simulink model "sm_tracked_vehicle_belt"  (R2025a)
settings: Solver=ode23t  StartTime=0.0  StopTime=50  MaxStep=0.01  RelTol=1e-4  AbsTol=1e-5  EnableMultiTasking=on
PreLoadFcn:
  | sm_tracked_vehicle_belt_param
StartFcn:
  | tic;
StopFcn:
  | Elapsed_Sim_Time = toc;
  | disp(['Elapsed Sim Time = ' num2str(Elapsed_Sim_Time)]);
undefined symbols (not defined in the file): belt, roller, vehbody, X, Y, Z
libraries: sm_lib x9, nesl_utility x3, SCF_Custom_Forces_lib x2, simulink x2, sm_tracked_vehicle_belt_lib x2, Camera_Frame_Definitions x1
CloseFcn:
  | try,close(h1_sm_tread_drive),end
  | clear h1_sm_tread_drive
  | 
  | clear logsout_sm_tread_drive
  | clear simlog_sm_tread_drive
Description:
  | Tread Drive on Uneven Surface
  | 
  | Copyright 2018-2026 The MathWorks, Inc.
settings Model: Creator=smiller  LastModifiedBy=smiller
settings SolverCC: AutoScaleAbsTol=off  AlgebraicLoopSolver=TrustRegion
settings DataIOCC: SaveFormat=Array  ReturnWorkspaceOutputs=off  SignalLoggingName=logsout_sm_tracked_vehicle_belt
settings OptimizationCC: ReuseModelBlockBuffer=off  LifeSpan=inf
settings DebuggingCC: SolverPrmCheckMsg=warning  UnconnectedInputMsg=warning  UnconnectedLineMsg=warning  AllowSymbolicDim=off  PregeneratedLibrarySubsystemCodeDiagnostic=none  SFUnexpectedBacktrackingDiag=warning  SFNoUnconditionalDefaultTransitionDiag=warning  SFExecutionAtInitializationDiag=none  ArithmeticOperatorsInVariantConditions=warning
settings HardwareCC: ProdBitPerPointer=32.0  ProdBitPerSizeT=32.0  ProdBitPerPtrDiffT=32.0  ProdLargestAtomicFloat=None  ProdIntDivRoundTo=Undefined  ProdEndianess=Unspecified  ProdWordSize=32.0  ProdHWDeviceType=32-bit Generic
settings ModelReferenceCC: EnableRefExpFcnMdlSchedulingChecks=on  PropagateSignalLabelsOutOfModel=off
settings SFSimCC: SimUseLocalCustomCode=off  CustomCodeUndefinedFunction=UseInterfaceOnly
settings RTWCC: RTWUseLocalCustomCode=off  GPUComputeCapability=3.5  DLArmComputeVersion=19.05
settings CodeAppCC: StateflowObjectComments=on
settings GRTTargetCC: TargetLangStandard=C89/C90 (ANSI)
settings ConfigComp: CovMetricSettings=dw  CovSaveCumulativeToWorkspaceVar=on  CovSaveSingleToWorkspaceVar=on  CovExternalEMLEnable=off  CovSFcnEnable=off
settings SimscapeCC: SimscapeNormalizeSystem=off  SimscapeLogType=all  SimscapeLogSimulationStatistics=on  SimscapeLogName=simlog_sm_tracked_vehicle_belt  SimscapeLogLimitData=off  SimscapeLogDataHistory=20000.0
settings ConfigurationSet: Description=SimMechanics 2G
settings DiagnosticsConfigSet: SimMechanicsConflictingReferenceFrames=none  SimMechanicsRigidlyBoundBlock=none
settings ExplorerConfigSet: InternalSimMechanicsExplorerSettings="<ExplorerConfiguration><canonicalview>default</canonicalview><AnimationSetting><BasePlaybackSpeed>1.0</BasePlaybackSpeed><PlaybackSpeedFactor>2.0</PlaybackSpeedFactor></AnimationSetting><TilePanel><TileInfo><Tiles Columns=\"2\" Count=\"3\" Rows=\"2\"><Column Weight=\"0.4996\"/><Column Weight=\"0.5004\"/><Row Weight=\"0.6676\"/><Row Weight=\"0.3324\"/><Tile Height=\"2\" Width=\"1\" X=\"0\" Y=\"0\"/><Tile Height=\"1\" Width=\"1\" X=\"1\" Y=\"0\"/><Tile Height=\"1\" Width=\"1\" X=\"1\" Y=\"1\"/></Tiles></TileInfo><SceneInfo><SceneViewer><BGColor><R>1</R><G>1</G><B>1</B></BGColor><Camera><DoPerspective>on</DoPerspective><Position><X>1.93552410841574951</X><Y>-22.2249086507629947</Y><Z>1.90260789180906764</Z></Position><Center><X>1.18525502751870504</X><Y>-21.5996844166821234</Y><Z>1.68768706134376867</Z></Center><Up><X>-0.16510675539218278</X><Y>0.137588962826818928</Y><Z>0.976631474319820447</Z></Up><ViewLimDist>1</ViewLimDist><YLim>0.466307658154998583</YLim><XLim>0.425934700738981431</XLim></Camera></SceneViewer><SceneViewer><BGColor><R>1</R><G>1</G><B>1</B></BGColor><Camera><DoPerspective>off</DoPerspective><Position><X>9.13279417173888497</X><Y>-10.8073529611331143</Y><Z>295.016351338458605</Z></Position><Center><X>9.13279417173888497</X><Y>-10.8073529611331143</Y><Z>-0.0192398869523913163</Z></Center><Up><X>0</X><Y>1</Y><Z>-0</Z></Up><ViewLimDist>1</ViewLimDist><YLim>13.4087479739997679</YLim><XLim>18.561454619030247</XLim></Camera></SceneViewer><SceneViewer><BGColor><R>1</R><G>1</G><B>1</B></BGColor><Camera><DoPerspective>on</DoPerspective><Position><X>3.00605602641301672</X><Y>-17.9535217836110448</Y><Z>1.77667486241447481</Z></Position><Center><X>2.04688726115486386</X><Y>-18.1627945947119365</Y><Z>1.58641143900608261</Z></Center><Up><X>-0.185488496866644897</X><Y>-0.0423982058506443826</Y><Z>0.981731332733553508</Z></Up><ViewLimDist>1</ViewLimDist><YLim>0.466307658154998583</YLim><XLim>1.30813741270030581</XLim></Camera></SceneViewer></SceneInfo></TilePanel><MechEditorPanel><Cameras><Camera><Id>Camera1</Id><Value><Name>Track FixO FR</Name><NativeCamera><PositionTrackingFeature>Camera_Frames.Frame_FixO_FR.R</PositionTrackingFeature><CenterTrackingFeature>Camera_Frames.Frame_FixO_FR.R</CenterTrackingFeature><UpVectorTrackingFeature>Camera_Frames.Frame_FixO_FR.R</UpVectorTrackingFeature><CenterTrackingOrigin>off</CenterTrackingOrigin><CenterTrackingDirection>+X</CenterTrackingDirection><UpVectorTrackingDirection>+Z</UpVectorTrackingDirection></NativeCamera></Value></Camera><Camera><Id>Camera2</Id><Value><Name>Track FixO Right</Name><NativeCamera><PositionTrackingFeature>Camera_Frames.Frame_FixO_Right.R</PositionTrackingFeature><CenterTrackingFeature>Camera_Frames.Frame_FixO_Right.R</CenterTrackingFeature><UpVectorTrackingFeature>Camera_Frames.Frame_FixO_Right.R</UpVectorTrackingFeature><CenterTrackingOrigin>off</CenterTrackingOrigin><CenterTrackingDirection>+X</CenterTrackingDirection><UpVectorTrackingDirection>+Z</UpVectorTrackingDirection></NativeCamera></Value></Camera><Camera><Id>Camera3</Id><Value><Name>Track FixO RR</Name><NativeCamera><PositionTrackingFeature>Camera_Frames.Frame_FixO_RR.R</PositionTrackingFeature><CenterTrackingFeature>Camera_Frames.Frame_FixO_RR.R</CenterTrackingFeature><UpVectorTrackingFeature>Camera_Frames.Frame_FixO_RR.R</UpVectorTrackingFeature><CenterTrackingOrigin>off</CenterTrackingOrigin><CenterTrackingDirection>+X</CenterTrackingDirection><UpVectorTrackingDirection>+Z</UpVectorTrackingDirection></NativeCamera></Value></Camera><Camera><Id>Camera4</Id><Value><Name>Track FixO RL</Name><NativeCamera><PositionTrackingFeature>Camera_Frames.Frame_FixO_RL.R</PositionTrackingFeature><CenterTrackingFeature>Camera_Frames.Frame_FixO_RL.R</CenterTrackingFeature><UpVectorTrackingFeature>Camera_Frames.Frame_FixO_RL.R</UpVectorTrackingFeature><CenterTrackingOrigin>off</CenterTrackingOrigin><CenterTrackingDirection>+X</CenterTrackingDirection><UpVectorTrackingDirection>+Z</UpVectorTrackingDirection></NativeCamera></Value></Camera><Camera><Id>Camera5</Id><Value><Name>Track FixO Left</Name><NativeCamera><PositionTrackingFeature>Camera_Frames.Frame_FixO_Left.R</PositionTrackingFeature><CenterTrackingFeature>Camera_Frames.Frame_FixO_Left.R</CenterTrackingFeature><UpVectorTrackingFeature>Camera_Frames.Frame_FixO_Left.R</UpVectorTrackingFeature><CenterTrackingOrigin>off</CenterTrackingOrigin><CenterTrackingDirection>+X</CenterTrackingDirection><UpVectorTrackingDirection>+Z</UpVectorTrackingDirection></NativeCamera></Value></Camera><Camera><Id>Camera6</Id><Value><Name>Track FixO FL</Name><NativeCamera><PositionTrackingFeature>Camera_Frames.Frame_FixO_FL.R</PositionTrackingFeature><CenterTrackingFeature>Camera_Frames.Frame_FixO_FL.R</CenterTrackingFeature><UpVectorTrackingFeature>Camera_Frames.Frame_FixO_FL.R</UpVectorTrackingFeature><CenterTrackingOrigin>off</CenterTrackingOrigin><CenterTrackingDirection>+X</CenterTrackingDirection><UpVectorTrackingDirection>+Z</UpVectorTrackingDirection></NativeCamera></Value></Camera><Camera><Id>Camera7</Id><Value><Name>Track FixO Top</Name><NativeCamera><PositionTrackingFeature>Camera_Frames.Frame_FixO_Top.R</PositionTrackingFeature><CenterTrackingFeature>Camera_Frames.Frame_FixO_Top.R</CenterTrackingFeature><UpVectorTrackingFeature>Camera_Frames.Frame_FixO_Top.R</UpVectorTrackingFeature><CenterTrackingOrigin>off</CenterTrackingOrigin><CenterTrackingDirection>+X</CenterTrackingDirection><UpVectorTrackingDirection>+Z</UpVectorTrackingDirection></NativeCamera></Value></Camera><Camera><Id>Camera8</Id><Value><Name>Track FixO Front</Name><NativeCamera><PositionTrackingFeature>Camera_Frames.Frame_FixO_Front.R</PositionTrackingFeature><CenterTrackingFeature>Camera_Frames.Frame_FixO_Front.R</CenterTrackingFeature><UpVectorTrackingFeature>Camera_Frames.Frame_FixO_Front.R</UpVectorTrackingFeature><CenterTrackingOrigin>off</CenterTrackingOrigin><CenterTrackingDirection>+X</CenterTrackingDirection><UpVectorTrackingDirection>+Z</UpVectorTrackingDirection></NativeCamera></Value></Camera><Camera><Id>Camera9</Id><Value><Name>Track FixO Rear</Name><NativeCamera><PositionTrackingFeature>Camera_Frames.Frame_FixO_Rear.R</PositionTrackingFeature><CenterTrackingFeature>Camera_Frames.Frame_FixO_Rear.R</CenterTrackingFeature><UpVectorTrackingFeature>Camera_Frames.Frame_FixO_Rear.R</UpVectorTrackingFeature><CenterTrackingOrigin>off</CenterTrackingOrigin><CenterTrackingDirection>+X</CenterTrackingDirection><UpVectorTrackingDirection>+Z</UpVectorTrackingDirection></NativeCamera></Value></Camera><Camera><Id>Camera10</Id><Value><Name>Track FR</Name><NativeCamera><PositionTrackingFeature>Camera_Frames.Frame_FR.R</PositionTrackingFeature><CenterTrackingFeature>Camera_Frames.Frame_FR.R</CenterTrackingFeature><UpVectorTrackingFeature>Camera_Frames.Frame_FR.R</UpVectorTrackingFeature><CenterTrackingOrigin>off</CenterTrackingOrigin><CenterTrackingDirection>+X</CenterTrackingDirection><UpVectorTrackingDirection>+Z</UpVectorTrackingDirection></NativeCamera></Value></Camera><Camera><Id>Camera11</Id><Value><Name>Track Right</Name><NativeCamera><PositionTrackingFeature>Camera_Frames.Frame_Right.R</PositionTrackingFeature><CenterTrackingFeature>Camera_Frames.Frame_Right.R</CenterTrackingFeature><UpVectorTrackingFeature>Camera_Frames.Frame_Right.R</UpVectorTrackingFeature><CenterTrackingOrigin>off</CenterTrackingOrigin><CenterTrackingDirection>+X</CenterTrackingDirection><UpVectorTrackingDirection>+Z</UpVectorTrackingDirection></NativeCamera></Value></Camera><Camera><Id>Camera12</Id><Value><Name>Track RR</Name><NativeCamera><PositionTrackingFeature>Camera_Frames.Frame_RR.R</PositionTrackingFeature><CenterTrackingFeature>Camera_Frames.Frame_RR.R</CenterTrackingFeature><UpVectorTrackingFeature>Camera_Frames.Frame_RR.R</UpVectorTrackingFeature><CenterTrackingOrigin>off</CenterTrackingOrigin><CenterTrackingDirection>+X</CenterTrackingDirection><UpVectorTrackingDirection>+Z</UpVectorTrackingDirection></NativeCamera></Value></Camera><Camera><Id>Camera13</Id><Value><Name>Track RL</Name><NativeCamera><PositionTrackingFeature>Camera_Frames.Frame_RL.R</PositionTrackingFeature><CenterTrackingFeature>Camera_Frames.Frame_RL.R</CenterTrackingFeature><UpVectorTrackingFeature>Camera_Frames.Frame_RL.R</UpVectorTrackingFeature><CenterTrackingOrigin>off</CenterTrackingOrigin><CenterTrackingDirection>+X</CenterTrackingDirection><UpVectorTrackingDirection>+Z</UpVectorTrackingDirection></NativeCamera></Value></Camera><Camera><Id>Camera14</Id><Value><Name>Track Left</Name><NativeCamera><PositionTrackingFeature>Camera_Frames.Frame_Left.R</PositionTrackingFeature><CenterTrackingFeature>Camera_Frames.Frame_Left.R</CenterTrackingFeature><UpVectorTrackingFeature>Camera_Frames.Frame_Left.R</UpVectorTrackingFeature><CenterTrackingOrigin>off</CenterTrackingOrigin><CenterTrackingDirection>+X</CenterTrackingDirection><UpVectorTrackingDirection>+Z</UpVectorTrackingDirection></NativeCamera></Value></Camera><Camera><Id>Camera15</Id><Value><Name>Track FL</Name><NativeCamera><PositionTrackingFeature>Camera_Frames.Frame_FL.R</PositionTrackingFeature><CenterTrackingFeature>Camera_Frames.Frame_FL.R</CenterTrackingFeature><UpVectorTrackingFeature>Camera_Frames.Frame_FL.R</UpVectorTrackingFeature><CenterTrackingOrigin>off</CenterTrackingOrigin><CenterTrackingDirection>+X</CenterTrackingDirection><UpVectorTrackingDirection>+Z</UpVectorTrackingDirection></NativeCamera></Value></Camera><Camera><Id>Camera16</Id><Value><Name>Track Top</Name><NativeCamera><PositionTrackingFeature>Camera_Frames.Frame_Top.R</PositionTrackingFeature><CenterTrackingFeature>Camera_Frames.Frame_Top.R</CenterTrackingFeature><UpVectorTrackingFeature>Camera_Frames.Frame_Top.R</UpVectorTrackingFeature><CenterTrackingOrigin>off</CenterTrackingOrigin><CenterTrackingDirection>+X</CenterTrackingDirection><UpVectorTrackingDirection>+Z</UpVectorTrackingDirection></NativeCamera></Value></Camera><Camera><Id>Camera17</Id><Value><Name>Track Front</Name><NativeCamera><PositionTrackingFeature>Camera_Frames.Frame_Front.R</PositionTrackingFeature><CenterTrackingFeature>Camera_Frames.Frame_Front.R</CenterTrackingFeature><UpVectorTrackingFeature>Camera_Frames.Frame_Front.R</UpVectorTrackingFeature><CenterTrackingOrigin>off</CenterTrackingOrigin><CenterTrackingDirection>+X</CenterTrackingDirection><UpVectorTrackingDirection>+Z</UpVectorTrackingDirection></NativeCamera></Value></Camera><Camera><Id>Camera18</Id><Value><Name>Track Rear</Name><NativeCamera><PositionTrackingFeature>Camera_Frames.Frame_Rear.R</PositionTrackingFeature><CenterTrackingFeature>Camera_Frames.Frame_Rear.R</CenterTrackingFeature><UpVectorTrackingFeature>Camera_Frames.Frame_Rear.R</UpVectorTrackingFeature><CenterTrackingOrigin>off</CenterTrackingOrigin><CenterTrackingDirection>+X</CenterTrackingDirection><UpVectorTrackingDirection>+Z</UpVectorTrackingDirection></NativeCamera></Value></Camera><Camera><Id>Camera19</Id><Value><Name>Track SuspF</Name><NativeCamera><PositionTrackingFeature>Camera_Frames.Frame_SuspF.R</PositionTrackingFeature><CenterTrackingFeature>Camera_Frames.Frame_SuspF.R</CenterTrackingFeature><UpVectorTrackingFeature>Camera_Frames.Frame_SuspF.R</UpVectorTrackingFeature><CenterTrackingOrigin>off</CenterTrackingOrigin><CenterTrackingDirection>+X</CenterTrackingDirection><UpVectorTrackingDirection>+Z</UpVectorTrackingDirection></NativeCamera></Value></Camera><Camera><Id>Camera20</Id><Value><Name>Track SuspR</Name><NativeCamera><PositionTrackingFeature>Camera_Frames.Frame_SuspR.R</PositionTrackingFeature><CenterTrackingFeature>Camera_Frames.Frame_SuspR.R</CenterTrackingFeature><UpVectorTrackingFeature>Camera_Frames.Frame_SuspR.R</UpVectorTrackingFeature><CenterTrackingOrigin>off</CenterTrackingOrigin><CenterTrackingDirection>+X</CenterTrackingDirection><UpVectorTrackingDirection>+Z</UpVectorTrackingDirection></NativeCamera></Value></Camera><Camera><Id>Camera21</Id><Value><Name>Track WheelFR</Name><NativeCamera><PositionTrackingFeature>Camera_Frames.Frame_Wheel_FR.R</PositionTrackingFeature><CenterTrackingFeature>Camera_Frames.Frame_Wheel_FR.R</CenterTrackingFeature><UpVectorTrackingFeature>Camera_Frames.Frame_Wheel_FR.R</UpVectorTrackingFeature><CenterTrackingOrigin>off</CenterTrackingOrigin><CenterTrackingDirection>+X</CenterTrackingDirection><UpVectorTrackingDirection>+Z</UpVectorTrackingDirection></NativeCamera></Value></Camera><Camera><Id>Camera22</Id><Value><Name>Track WheelRR</Name><NativeCamera><PositionTrackingFeature>Camera_Frames.Frame_Wheel_RR.R</PositionTrackingFeature><CenterTrackingFeature>Camera_Frames.Frame_Wheel_RR.R</CenterTrackingFeature><UpVectorTrackingFeature>Camera_Frames.Frame_Wheel_RR.R</UpVectorTrackingFeature><CenterTrackingOrigin>off</CenterTrackingOrigin><CenterTrackingDirection>+X</CenterTrackingDirection><UpVectorTrackingDirection>+Z</UpVectorTrackingDirection></NativeCamera></Value></Camera><Camera><Id>Camera23</Id><Value><Name>Track WheelRL</Name><NativeCamera><PositionTrackingFeature>Camera_Frames.Frame_Wheel_RL.R</PositionTrackingFeature><CenterTrackingFeature>Camera_Frames.Frame_Wheel_RL.R</CenterTrackingFeature><UpVectorTrackingFeature>Camera_Frames.Frame_Wheel_RL.R</UpVectorTrackingFeature><CenterTrackingOrigin>off</CenterTrackingOrigin><CenterTrackingDirection>+X</CenterTrackingDirection><UpVectorTrackingDirection>+Z</UpVectorTrackingDirection></NativeCamera></Value></Camera><Camera><Id>Camera24</Id><Value><Name>Track WheelFL</Name><NativeCamera><PositionTrackingFeature>Camera_Frames.Frame_Wheel_FL.R</PositionTrackingFeature><CenterTrackingFeature>Camera_Frames.Frame_Wheel_FL.R</CenterTrackingFeature><UpVectorTrackingFeature>Camera_Frames.Frame_Wheel_FL.R</UpVectorTrackingFeature><CenterTrackingOrigin>off</CenterTrackingOrigin><CenterTrackingDirection>+X</CenterTrackingDirection><UpVectorTrackingDirection>+Z</UpVectorTrackingDirection></NativeCamera></Value></Camera><Camera><Id>Camera25</Id><Value><Name>View Seat FL</Name><NativeCamera><PositionTrackingFeature>Camera_Frames.Frame_View_Seat_FL.R</PositionTrackingFeature><CenterTrackingFeature>Camera_Frames.Frame_View_Seat_FL.R</CenterTrackingFeature><UpVectorTrackingFeature>Camera_Frames.Frame_View_Seat_FL.R</UpVectorTrackingFeature><CenterTrackingOrigin>off</CenterTrackingOrigin><CenterTrackingDirection>+X</CenterTrackingDirection><UpVectorTrackingDirection>+Z</UpVectorTrackingDirection></NativeCamera></Value></Camera><Camera><Id>Camera26</Id><Value><Name>View Seat FR</Name><NativeCamera><PositionTrackingFeature>Camera_Frames.Frame_View_Seat_FR.R</PositionTrackingFeature><CenterTrackingFeature>Camera_Frames.Frame_View_Seat_FR.R</CenterTrackingFeature><UpVectorTrackingFeature>Camera_Frames.Frame_View_Seat_FR.R</UpVectorTrackingFeature><CenterTrackingOrigin>off</CenterTrackingOrigin><CenterTrackingDirection>+X</CenterTrackingDirection><UpVectorTrackingDirection>+Z</UpVectorTrackingDirection></NativeCamera></Value></Camera><Camera><Id>Camera27</Id><Value><Name>View Susp FR</Name><NativeCamera><PositionTrackingFeature>Camera_Frames.Frame_View_Susp_FR.R</PositionTrackingFeature><CenterTrackingFeature>Camera_Frames.Frame_View_Susp_FR.R</CenterTrackingFeature><UpVectorTrackingFeature>Camera_Frames.Frame_View_Susp_FR.R</UpVectorTrackingFeature><CenterTrackingOrigin>off</CenterTrackingOrigin><CenterTrackingDirection>+X</CenterTrackingDirection><UpVectorTrackingDirection>+Z</UpVectorTrackingDirection></NativeCamera></Value></Camera><Camera><Id>Camera28</Id><Value><Name>View Susp RR</Name><NativeCamera><PositionTrackingFeature>Camera_Frames.Frame_View_Susp_RR.R</PositionTrackingFeature><CenterTrackingFeature>Camera_Frames.Frame_View_Susp_RR.R</CenterTrackingFeature><UpVectorTrackingFeature>Camera_Frames.Frame_View_Susp_RR.R</UpVectorTrackingFeature><CenterTrackingOrigin>off</CenterTrackingOrigin><CenterTrackingDirection>+X</CenterTrackingDirection><UpVectorTrackingDirection>+Z</UpVectorTrackingDirection></NativeCamera></Value></Camera><Camera><Id>Camera29</Id><Value><Name>View Susp RL</Name><NativeCamera><PositionTrackingFeature>Camera_Frames.Frame_View_Susp_RL.R</PositionTrackingFeature><CenterTrackingFeature>Camera_Frames.Frame_View_Susp_RL.R</CenterTrackingFeature><UpVectorTrackingFeature>Camera_Frames.Frame_View_Susp_RL.R</UpVectorTrackingFeature><CenterTrackingOrigin>off</CenterTrackingOrigin><CenterTrackingDirection>+X</CenterTrackingDirection><UpVectorTrackingDirection>+Z</UpVectorTrackingDirection></NativeCamera></Value></Camera><Camera><Id>Camera30</Id><Value><Name>View Susp FL</Name><NativeCamera><PositionTrackingFeature>Camera_Frames.Frame_View_Susp_FL.R</PositionTrackingFeature><CenterTrackingFeature>Camera_Frames.Frame_View_Susp_FL.R</CenterTrackingFeature><UpVectorTrackingFeature>Camera_Frames.Frame_View_Susp_FL.R</UpVectorTrackingFeature><CenterTrackingOrigin>off</CenterTrackingOrigin><CenterTrackingDirection>+X</CenterTrackingDirection><UpVectorTrackingDirection>+Z</UpVectorTrackingDirection></NativeCamera></Value></Camera><Camera><Id>Camera31</Id><Value><Name>Dolly Camera</Name><NativeCamera><PositionTrackingFeature>Camera_Frames.Frame_Dolly.R</PositionTrackingFeature><CenterTrackingFeature>Camera_Frames.Frame_Dolly.R</CenterTrackingFeature><UpVectorTrackingFeature>Camera_Frames.Frame_Dolly.R</UpVectorTrackingFeature><CenterTrackingOrigin>off</CenterTrackingOrigin><CenterTrackingDirection>+X</CenterTrackingDirection><UpVectorTrackingDirection>+Z</UpVectorTrackingDirection></NativeCamera></Value></Camera><Camera><Id>Camera32</Id><Value><Name>Track Dolly Camera</Name><NativeCamera><PositionTrackingFeature>Camera_Frames.Frame_Dolly.R</PositionTrackingFeature><CenterTrackingFeature>Camera_Frames.Transform_Camera_Ref.F</CenterTrackingFeature><UpVectorTrackingFeature>Camera_Frames.World_Frame.W</UpVectorTrackingFeature><CenterTrackingOrigin>on</CenterTrackingOrigin><UpVectorTrackingDirection>+Z</UpVectorTrackingDirection></NativeCamera></Value></Camera></Cameras><GfxPanelCameraMap><MapElement CameraMLId=\"Camera1\" GfxPanelIndex=\"0\"/><MapElement CameraMLId=\"Camera18\" GfxPanelIndex=\"2\"/></GfxPanelCameraMap><VideoCreator><PlaybackSpeedRatio>1.0</PlaybackSpeedRatio><FrameRate>30</FrameRate><VideoFormat>MPEG-4</VideoFormat><FrameSize>[800 450]</FrameSize></VideoCreator></MechEditorPanel></ExplorerConfiguration>"

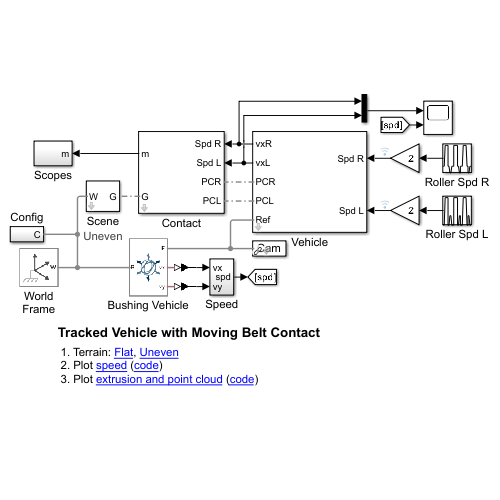
[thumbnail: Simulink's stored preview of the top-level diagram]
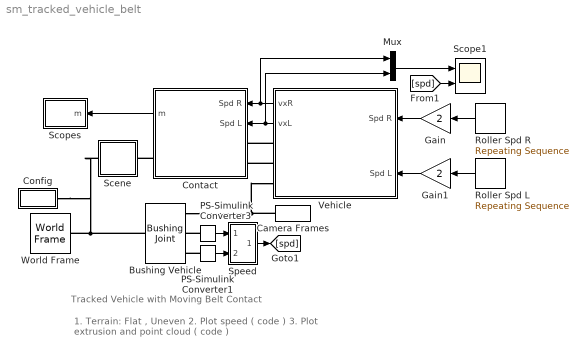
== system sm_tracked_vehicle_belt ==
  note: 1. Terrain: Flat , Uneven
      | 2. Plot speed ( code )
      | 3. Plot extrusion and point cloud ( code )
  note: Tracked Vehicle with Moving Belt Contact
  Bushing Vehicle : sm_lib/Joints/Bushing Joint  JointMode=Normal  CompositeWrenchDir=FollowerOnBase  CompositeWrenchFrame=BaseFrame  SenseConstraintForce=off  SenseConstraintTorque=off  SenseTotalForce=off  SenseTotalTorque=off  PxPositionTargetSpecify=on  PxPositionTargetPriority=High  PxPositionTargetValue=vehbody.x0  PxPositionTargetValueUnits=m  PxVelocityTargetSpecify=off  PxVelocityTargetPriority=High  PxVelocityTargetValue=0  PxVelocityTargetValueUnits=m/s  PxEquilibriumPosition=0  PxEquilibriumPositionUnits=m  PxSpringStiffness=0  PxSpringStiffnessUnits=N/m  PxDampingCoefficient=1  PxDampingCoefficientUnits=N/(m/s)  PxLowerLimitSpecify=off  PxLowerLimitBound=-1  PxLowerLimitBoundUnits=m  PxLowerLimitStiffness=1e6  PxLowerLimitStiffnessUnits=N/m  PxLowerLimitDamping=1e3  PxLowerLimitDampingUnits=N/(m/s)  PxLowerLimitTransitionRegionWidth=1e-4  PxLowerLimitTransitionRegionWidthUnits=m  PxUpperLimitSpecify=off  PxUpperLimitBound=1  PxUpperLimitBoundUnits=m  PxUpperLimitStiffness=1e6  PxUpperLimitStiffnessUnits=N/m  PxUpperLimitDamping=1e3  PxUpperLimitDampingUnits=N/(m/s)  PxUpperLimitTransitionRegionWidth=1e-4  PxUpperLimitTransitionRegionWidthUnits=m  PxTorqueActuationMode=NoTorque  PxMotionActuationMode=ComputedMotion  PxSensePosition=off  PxSenseVelocity=on  PxSenseAcceleration=off  PxSenseTorqueForce=off  PxSenseLowerLimitTorqueForce=off  PxSenseUpperLimitTorqueForce=off  PyPositionTargetSpecify=on  PyPositionTargetPriority=High  PyPositionTargetValue=0  PyPositionTargetValueUnits=m  PyVelocityTargetSpecify=off  PyVelocityTargetPriority=High  PyVelocityTargetValue=0  PyVelocityTargetValueUnits=m/s  PyEquilibriumPosition=0  PyEquilibriumPositionUnits=m  PySpringStiffness=0  PySpringStiffnessUnits=N/m  PyDampingCoefficient=1  PyDampingCoefficientUnits=N/(m/s)  PyLowerLimitSpecify=off  PyLowerLimitBound=-1  PyLowerLimitBoundUnits=m  PyLowerLimitStiffness=1e6  PyLowerLimitStiffnessUnits=N/m  PyLowerLimitDamping=1e3  PyLowerLimitDampingUnits=N/(m/s)  PyLowerLimitTransitionRegionWidth=1e-4  PyLowerLimitTransitionRegionWidthUnits=m  PyUpperLimitSpecify=off  PyUpperLimitBound=1  PyUpperLimitBoundUnits=m  PyUpperLimitStiffness=1e6  PyUpperLimitStiffnessUnits=N/m  PyUpperLimitDamping=1e3  PyUpperLimitDampingUnits=N/(m/s)  PyUpperLimitTransitionRegionWidth=1e-4  PyUpperLimitTransitionRegionWidthUnits=m  PyTorqueActuationMode=NoTorque  PyMotionActuationMode=ComputedMotion  PySensePosition=off  PySenseVelocity=on  PySenseAcceleration=off  PySenseTorqueForce=off  PySenseLowerLimitTorqueForce=off  PySenseUpperLimitTorqueForce=off  PzPositionTargetSpecify=on  PzPositionTargetPriority=High  PzPositionTargetValue=vehbody.z0  PzPositionTargetValueUnits=m  PzVelocityTargetSpecify=off  PzVelocityTargetPriority=High  PzVelocityTargetValue=0  PzVelocityTargetValueUnits=m/s  PzEquilibriumPosition=0  PzEquilibriumPositionUnits=m  PzSpringStiffness=0  PzSpringStiffnessUnits=N/m  PzDampingCoefficient=0  PzDampingCoefficientUnits=N/(m/s)  PzLowerLimitSpecify=off  PzLowerLimitBound=-1  PzLowerLimitBoundUnits=m  PzLowerLimitStiffness=1e6  PzLowerLimitStiffnessUnits=N/m  PzLowerLimitDamping=1e3  PzLowerLimitDampingUnits=N/(m/s)  PzLowerLimitTransitionRegionWidth=1e-4  PzLowerLimitTransitionRegionWidthUnits=m  PzUpperLimitSpecify=off  PzUpperLimitBound=1  PzUpperLimitBoundUnits=m  PzUpperLimitStiffness=1e6  PzUpperLimitStiffnessUnits=N/m  PzUpperLimitDamping=1e3  PzUpperLimitDampingUnits=N/(m/s)  PzUpperLimitTransitionRegionWidth=1e-4  PzUpperLimitTransitionRegionWidthUnits=m  PzTorqueActuationMode=NoTorque  PzMotionActuationMode=ComputedMotion  PzSensePosition=off  PzSenseVelocity=off  PzSenseAcceleration=off  PzSenseTorqueForce=off  PzSenseLowerLimitTorqueForce=off  PzSenseUpperLimitTorqueForce=off  RxPositionTargetSpecify=on  RxPositionTargetPriority=High  RxPositionTargetValue=0  RxPositionTargetValueUnits=deg  RxVelocityTargetSpecify=off  RxVelocityTargetPriority=High  RxVelocityTargetValue=0  RxVelocityTargetValueUnits=deg/s  RxEquilibriumPosition=0  RxEquilibriumPositionUnits=deg  RxSpringStiffness=0  RxSpringStiffnessUnits=N*m/deg  RxDampingCoefficient=0  RxDampingCoefficientUnits=N*m/(deg/s)  RxLowerLimitSpecify=off  RxLowerLimitBound=-90  RxLowerLimitBoundUnits=deg  RxLowerLimitStiffness=1e4  RxLowerLimitStiffnessUnits=N*m/deg  RxLowerLimitDamping=10  RxLowerLimitDampingUnits=N*m/(deg/s)  RxLowerLimitTransitionRegionWidth=0.1  RxLowerLimitTransitionRegionWidthUnits=deg  RxUpperLimitSpecify=off  RxUpperLimitBound=90  RxUpperLimitBoundUnits=deg  RxUpperLimitStiffness=1e4  RxUpperLimitStiffnessUnits=N*m/deg  RxUpperLimitDamping=10  RxUpperLimitDampingUnits=N*m/(deg/s)  RxUpperLimitTransitionRegionWidth=0.1  RxUpperLimitTransitionRegionWidthUnits=deg  RxTorqueActuationMode=NoTorque  RxMotionActuationMode=ComputedMotion  RxSensePosition=off  RxSenseVelocity=off  RxSenseAcceleration=off  RxSenseTorqueForce=off  RxSenseLowerLimitTorqueForce=off  RxSenseUpperLimitTorqueForce=off  RyPositionTargetSpecify=on  RyPositionTargetPriority=High  RyPositionTargetValue=0  RyPositionTargetValueUnits=deg  RyVelocityTargetSpecify=off  RyVelocityTargetPriority=High  RyVelocityTargetValue=0  RyVelocityTargetValueUnits=deg/s  RyEquilibriumPosition=0  RyEquilibriumPositionUnits=deg  RySpringStiffness=0  RySpringStiffnessUnits=N*m/deg  RyDampingCoefficient=0  RyDampingCoefficientUnits=N*m/(deg/s)  RyLowerLimitSpecify=off  RyLowerLimitBound=-90  RyLowerLimitBoundUnits=deg  RyLowerLimitStiffness=1e4  RyLowerLimitStiffnessUnits=N*m/deg  RyLowerLimitDamping=10  RyLowerLimitDampingUnits=N*m/(deg/s)  RyLowerLimitTransitionRegionWidth=0.1  RyLowerLimitTransitionRegionWidthUnits=deg  RyUpperLimitSpecify=off  RyUpperLimitBound=90  RyUpperLimitBoundUnits=deg  RyUpperLimitStiffness=1e4  RyUpperLimitStiffnessUnits=N*m/deg  RyUpperLimitDamping=10  RyUpperLimitDampingUnits=N*m/(deg/s)  RyUpperLimitTransitionRegionWidth=0.1  RyUpperLimitTransitionRegionWidthUnits=deg  RyTorqueActuationMode=NoTorque  RyMotionActuationMode=ComputedMotion  RySensePosition=off  RySenseVelocity=off  RySenseAcceleration=off  RySenseTorqueForce=off  RySenseLowerLimitTorqueForce=off  RySenseUpperLimitTorqueForce=off  RzPositionTargetSpecify=off  RzPositionTargetPriority=High  RzPositionTargetValue=0  RzPositionTargetValueUnits=deg  RzVelocityTargetSpecify=off  RzVelocityTargetPriority=High  RzVelocityTargetValue=0  RzVelocityTargetValueUnits=deg/s  RzEquilibriumPosition=0  RzEquilibriumPositionUnits=deg  RzSpringStiffness=0  RzSpringStiffnessUnits=N*m/deg  RzDampingCoefficient=0  RzDampingCoefficientUnits=N*m/(deg/s)  RzLowerLimitSpecify=off  RzLowerLimitBound=-90  RzLowerLimitBoundUnits=deg  RzLowerLimitStiffness=1e4  RzLowerLimitStiffnessUnits=N*m/deg  RzLowerLimitDamping=10  RzLowerLimitDampingUnits=N*m/(deg/s)  RzLowerLimitTransitionRegionWidth=0.1  RzLowerLimitTransitionRegionWidthUnits=deg  RzUpperLimitSpecify=off  RzUpperLimitBound=90  RzUpperLimitBoundUnits=deg  RzUpperLimitStiffness=1e4  RzUpperLimitStiffnessUnits=N*m/deg  RzUpperLimitDamping=10  RzUpperLimitDampingUnits=N*m/(deg/s)  RzUpperLimitTransitionRegionWidth=0.1  RzUpperLimitTransitionRegionWidthUnits=deg  RzTorqueActuationMode=NoTorque  RzMotionActuationMode=ComputedMotion  RzSensePosition=off  RzSenseVelocity=off  RzSenseAcceleration=off  RzSenseTorqueForce=off  RzSenseLowerLimitTorqueForce=off  RzSenseUpperLimitTorqueForce=off
  Camera Frames : Camera_Frame_Definitions/Camera Frames  Camera=Camera  popup_dolly_camera=XYZ
  Config : Subsystem
  Contact : Subsystem  mask(Contact Forces, Belts to Ground){k_collision=belt.ground.k, d_collision=belt.ground.b, d_width=belt.ground.twd, muk=belt.ground.muk, mus=belt.ground.mus, vth=belt.ground.vth}
      mask prompts: k_collision "Stiffness Coefficient (N/m)"; d_collision "Damping Coefficient (N/(m/s))"; d_width "Transition Region Width (m)"; muk "Coefficient of Kinetic Friction"; mus "Coefficient of Static Friction"; vth "Velocity Threshold"
      mask help: Models contact force between belts and ground. Translational speed of belt is an input to a custom force law that enables the belts to pull themselves across the surface.
      mask TypeOptions k_collision: Contact Track L/k_collision | Contact Track R/k_collision
      mask TypeOptions d_collision: Contact Track L/d_collision | Contact Track R/d_collision
      mask TypeOptions d_width: Contact Track L/d_width | Contact Track R/d_width
      mask TypeOptions muk: Contact Track L/muk | Contact Track R/muk
      mask TypeOptions mus: Contact Track L/mus | Contact Track R/mus
      mask TypeOptions vth: Contact Track L/vth | Contact Track R/vth
      mask DialogControl cont_normalForce Prompt: Normal Force
      mask DialogControl cont_frictionForce Prompt: Friction Force
  Gain : Gain  Gain=2
  Gain1 : Gain  Gain=2
  Mux : Mux  Inputs=2
  PS-Simulink Converter1 : nesl_utility/PS-Simulink Converter  PhysicalDomain=network_engine_domain  SubClassName=ps_output  LeftPortType=input  RightPortType=output  PseudoPeriodic=off  Frequencies=[]  VectorFormat=1-D array  Unit=1  AffineConversion=off
  PS-Simulink Converter3 : nesl_utility/PS-Simulink Converter  PhysicalDomain=network_engine_domain  SubClassName=ps_output  LeftPortType=input  RightPortType=output  PseudoPeriodic=off  Frequencies=[]  VectorFormat=1-D array  Unit=1  AffineConversion=off
  Roller Spd L : simulink/Sources/Repeating Sequence  rep_seq_t=[0 1 1.5 4.5 5 6 6.5 7.5 8 9]  rep_seq_y=[0 0 3 3 0 0 1 1 0 0]
  Roller Spd R : simulink/Sources/Repeating Sequence  rep_seq_t=[0 1 1.5 4.5 5 6 6.5 7.5 8 9]  rep_seq_y=[0 0 3 3 0 0 -1 -1 0 0]
  Scene : Subsystem  mask{popup_terrain=Uneven}
      mask prompts: popup_terrain "Terrain"
      mask init:
      | bh = gcb;
      | if(popup_terrain == 1)
      |     set_param([bh '/Grid Surface'],'ZHeights','Scene.Terrain.z_heights_data*0')
      | else
      |     set_param([bh '/Grid Surface'],'ZHeights','Scene.Terrain.z_heights_data')
      | end
      settings: AttributesFormatString=%<popup_terrain>
      mask TypeOptions popup_terrain: Flat | Uneven
  Scope1 : Scope  NumInputPorts=2
      settings: ActiveDisplayYMinimum=-0.88266  ActiveDisplayYMaximum=2.06398
  Scopes : Subsystem
  Speed : Subsystem
  Vehicle : Subsystem  mask{cyl_radius=roller.rad, cyl_density=roller.rho, cyl_color_custom=roller.clr, cyl_opacity=1, link_len=belt.l, link_xlen=belt.xlen, link_height=belt.h, link_rado=belt.rad, link_width=belt.w, link_mass=belt.m, link_opc=1, link_color=belt.clr, CoordinatesMatrix=belt.ptcld.pts, GraphicSphereRadius=belt.ptcld.rad, GraphicDiffuseColor=belt.ptcld.clr, GraphicOpacity=1, body_mass=vehbody.mass, track_sep=vehbody.tracksep}
      mask prompts: cyl_radius "Roller Radius (m)"; cyl_density "Density (kg/m^3)"; cyl_color_custom "Color [R G B] (0-1)"; cyl_opacity "Opacity (0-1)"; link_len "Sprocket-to-Idler (m)"; link_xlen "Center Roller x Position (0-1)"; link_height "Center Roller z Position (m)"; link_rado "Belt Outer Radius (m)"; link_width "Width (m)"; link_mass "Mass (kg)"; link_opc "Opacity (0-1)"; link_color "Color [R G B] (0-1)"; CoordinatesMatrix "Points [x y z] (m)"; GraphicSphereRadius "Radius (m)"; GraphicDiffuseColor "Color [R G B] (0-1)"; GraphicOpacity "Opacity (0-1)"; body_mass "Mass (kg)"; track_sep "Track Separation (m)"
      mask TypeOptions cyl_radius: Track L/cyl_radius | Track R/cyl_radius
      mask TypeOptions cyl_density: Track L/cyl_density | Track R/cyl_density
      mask TypeOptions cyl_color_custom: Track L/cyl_color_custom | Track R/cyl_color_custom
      mask TypeOptions cyl_opacity: Track L/cyl_opacity | Track R/cyl_opacity
      mask TypeOptions link_len: Track L/link_len | Track R/link_len
      mask TypeOptions link_xlen: Track L/link_xlen | Track R/link_xlen
      mask TypeOptions link_height: Track L/link_height | Track R/link_height
      mask TypeOptions link_rado: Track L/link_rado | Track R/link_rado | w to spd L/Gain | w to spd R/Gain
      mask TypeOptions link_width: Track L/link_width | Track R/link_width
      mask TypeOptions link_mass: Track L/link_mass | Track R/link_mass
      mask TypeOptions link_opc: Track L/link_opc | Track R/link_opc
      mask TypeOptions link_color: Track L/link_color | Track R/link_color
      mask TypeOptions CoordinatesMatrix: Track L/CoordinatesMatrix | Track R/CoordinatesMatrix
      mask TypeOptions GraphicSphereRadius: Track L/GraphicSphereRadius | Track R/GraphicSphereRadius
      mask TypeOptions GraphicDiffuseColor: Track L/GraphicDiffuseColor | Track R/GraphicDiffuseColor
      mask TypeOptions GraphicOpacity: Track L/GraphicOpacity | Track R/GraphicOpacity
      mask TypeOptions body_mass: Body/Mass
      mask DialogControl cont_roller Prompt: Roller
      mask DialogControl cont_belt Prompt: Belt
      mask DialogControl Container5 Prompt: Point Cloud
      mask DialogControl Container6 Prompt: Vehicle
  World Frame : sm_lib/Frames and Transforms/World Frame
  wires:
  PS-Simulink Converter3/1 -> Speed/1(vx)
  Roller Spd R/1 -> Gain/1
  Roller Spd L/1 -> Gain1/1
  PS-Simulink Converter1/1 -> Speed/2(vy)
  Speed/1(spd) -> [spd]
  Mux/1 -> Scope1/1
  Gain/1 -> Vehicle/1(Spd R)
  Gain1/1 -> Vehicle/2(Spd L)
  Contact/1(m) -> Scopes/1(m)
  Vehicle/1(vxR) -> Mux/1, Contact/1(Spd R)
  Vehicle/2(vxL) -> Mux/2, Contact/2(Spd L)
  [spd] -> Scope1/2
  connections:
  Bushing Vehicle/LConn1 -- Config/LConn1 -- Scene/LConn1 -- World Frame/RConn1
  Bushing Vehicle/RConn1 -- Vehicle/RConn3 -- Camera Frames/RConn1
  PS-Simulink Converter3/LConn1 -- Bushing Vehicle/RConn2
  Vehicle/RConn1 -- Contact/LConn1
  Vehicle/RConn2 -- Contact/LConn2
  PS-Simulink Converter1/LConn1 -- Bushing Vehicle/RConn3
  Contact/RConn1 -- Scene/RConn1

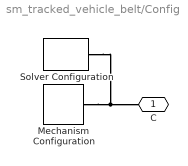
== system sm_tracked_vehicle_belt/Config ==
  Mechanism Configuration : sm_lib/Utilities/Mechanism Configuration  UniformGravity=Constant  GravityVector=[0 0 -9.80665]  GravityVectorUnits=m/s^2  LinearizationDelta=0.001  JointModeTransitionNonlinearIterations=2
  Solver Configuration : nesl_utility/Solver Configuration  PhysicalDomain=network_engine_domain  SubClassName=solver  LeftPortType=input  RightPortType=generic  Tones=[]  Harmonics=[]  SimulateNoise=off  Profile=off  UseLocalSampling=off  EnableSwitchedLinearOptims=on  FrequencyDomain=off  UseCCode=off  RelTol=0.001  AbsTol=1e-06  MinStep=1e-09  ToWorkspace=off  RevertToSquareIcSolve=off  NumHomotopyIterations=100  PhasorMode=off  PhasorModeNumHarmonics=1  ConsistencySolver=NEWTON_FTOL  IndexReductionMethod=DerivativeReplacement  DoDC=off  ResidualTolerance=1e-09  ConsistencyTolSource=GLOBAL  ConsistencyAbsTol=0.001  ConsistencyRelTol=0.001  ConsistencyTolFactor=0.001  UseLocalSolver=off  LocalSolverChoice=NE_BACKWARD_EULER_ADVANCER  ResolveIndetEquations=on  FunctionEvalNumThread=1  LocalSolverSampleTime=0.001  DoFixedCost=off  MaxNonlinIter=3  MaxModeIter=2  ComputeImpulses=off  ImpulseIterations=2  LinearAlgebra=Sparse  LinearAlgebraNumThread=0  EquationFormulation=NE_TIME_EF  DelaysMemoryBudget=1024  AutomaticFiltering=on  FilteringTimeConstant=0.001  PartitionStorageMethod=AS_NEEDED  PartitionMemoryBudget=1024  PartitionMethod=FAST  MultibodyUseLocalSolver=off  MultibodyLocalSolverChoice=ODE1  MultibodyLocalSolverSampleTime=0.001
  C : PMIOPort  Side=Left
  connections:
  Solver Configuration/RConn1 -- C/RConn1 -- Mechanism Configuration/RConn1

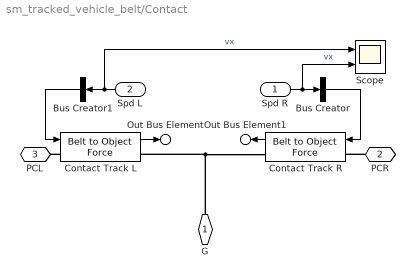
== system sm_tracked_vehicle_belt/Contact ==
  Spd R : Inport
  Spd L : Inport  Port=2
  Bus Creator : BusCreator  Inputs=1
  Bus Creator1 : BusCreator  Inputs=1
  Contact Track L : SCF_Custom_Forces_lib/Belt to Object Force  k_collision=k_collision  d_collision=d_collision  d_width=d_width  muk=muk  mus=mus  vth=vth
  Contact Track R : SCF_Custom_Forces_lib/Belt to Object Force  k_collision=k_collision  d_collision=d_collision  d_width=d_width  muk=muk  mus=mus  vth=vth
  Scope : Scope  NumInputPorts=2
      settings: ActiveDisplayYMinimum=-0.882  ActiveDisplayYMaximum=2.058  DataLoggingVariableName=ScopeData2
  G : PMIOPort  Side=Right
  PCR : PMIOPort  Port=2  Side=Left
  PCL : PMIOPort  Port=3  Side=Left
  Out Bus Element : Outport  PortName=m  Element=L
  Out Bus Element1 : Outport  PortName=m  Element=R
  wires:
  Bus Creator/1 -> Contact Track R/1
  Bus Creator1/1 -> Contact Track L/1
  Spd R/1 -> Scope/2, Bus Creator/1  "vx"
  Spd L/1 -> Scope/1, Bus Creator1/1  "vx"
  Contact Track L/1 -> Out Bus Element/1
  Contact Track R/1 -> Out Bus Element1/1
  connections:
  Contact Track L/LConn1 -- PCL/RConn1
  PCR/RConn1 -- Contact Track R/LConn1
  G/RConn1 -- Contact Track L/RConn1 -- Contact Track R/RConn1

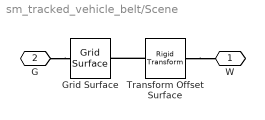
== system sm_tracked_vehicle_belt/Scene ==
  Grid Surface : sm_lib/Curves and Surfaces/Grid Surface  XGridVector=Scene.Terrain.xg  XGridVectorUnits=m  YGridVector=Scene.Terrain.yg  YGridVectorUnits=m  ZHeights=Scene.Terrain.z_heights_data  ZHeightsUnits=m  GraphicType=FromGeometry  GraphicVisPropType=SimpleVisualProperties  GraphicDiffuseColor=[0.8196 0.7255 0.5098]  GraphicOpacity=1.0  GraphicSpecularColor=[0.5 0.5 0.5 1.0]  GraphicAmbientColor=[0.15 0.15 0.15 1.0]  GraphicEmissiveColor=[0.0 0.0 0.0 1.0]  GraphicShininess=75
  Transform Offset Surface : sm_lib/Frames and Transforms/Rigid Transform  RotationMethod=None  FollAlignAxisA=+X  BaseAlignAxisA=+Y  FollAlignAxisB=+Y  BaseAlignAxisB=+Z  RotationStandardAxis=+Z  RotationAngle=0.0  RotationAngleUnits=deg  RotationArbitraryAxis=[0 0 1]  RotationSequenceAxes=FollowerAxes  RotationSequence=XYX  RotationSequenceAngles=[0 0 0]  RotationSequenceAnglesUnits=deg  RotationMatrix=[1 0 0; 0 1 0; 0 0 1]  Quaternion=[1 0 0 0]  TranslationMethod=Cartesian  TranslationCartesianOffset=[-20 -32 -1.3]  TranslationCartesianOffsetUnits=m  TranslationStandardAxis=+Z  TranslationStandardOffset=0  TranslationStandardOffsetUnits=m  TranslationROffset=0  TranslationROffsetUnits=m  TranslationThetaOffset=0  TranslationThetaOffsetUnits=deg  TranslationZOffset=0  TranslationZOffsetUnits=m
  W : PMIOPort  Side=Left
  G : PMIOPort  Port=2  Side=Right
  connections:
  Transform Offset Surface/RConn1 -- Grid Surface/LConn1
  Transform Offset Surface/LConn1 -- W/RConn1
  G/RConn1 -- Grid Surface/RConn1

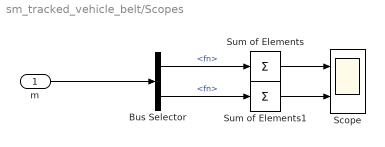
== system sm_tracked_vehicle_belt/Scopes ==
  m : Inport
  Bus Selector : BusSelector  OutputSignals=L.fn,R.fn
  Scope : Scope  NumInputPorts=2
      settings: ActiveDisplayYMinimum=-158668.51526  ActiveDisplayYMaximum=348701.73703
  Sum of Elements : Sum  Inputs=+
  Sum of Elements1 : Sum  Inputs=+
  wires:
  m/1 -> Bus Selector/1
  Bus Selector/1 -> Sum of Elements/1  "<fn>"
  Bus Selector/2 -> Sum of Elements1/1  "<fn>"
  Sum of Elements/1 -> Scope/1
  Sum of Elements1/1 -> Scope/2

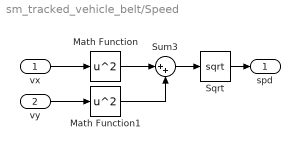
== system sm_tracked_vehicle_belt/Speed ==
  vx : Inport
  vy : Inport  Port=2
  Math Function : Math  Operator=square  SignedPower=on
  Math Function1 : Math  Operator=square  SignedPower=on
  Sqrt : Sqrt
  Sum3 : Sum  Inputs=|++
  spd : Outport
  wires:
  vx/1 -> Math Function/1
  Math Function1/1 -> Sum3/2
  vy/1 -> Math Function1/1
  Sum3/1 -> Sqrt/1
  Math Function/1 -> Sum3/1
  Sqrt/1 -> spd/1

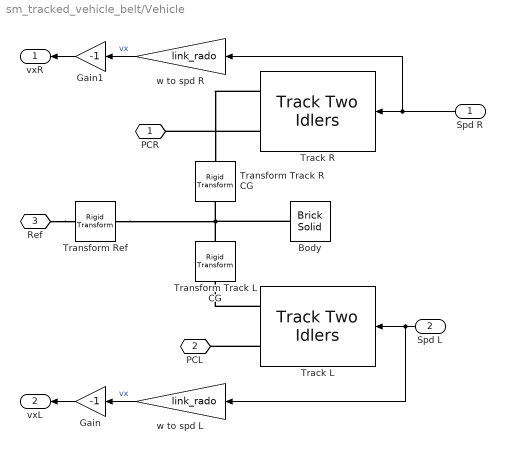
== system sm_tracked_vehicle_belt/Vehicle ==
  Spd R : Inport
  Spd L : Inport  Port=2
  Body : sm_lib/Body Elements/Brick Solid  BrickDimensions=[link_len/2 track_sep-link_width link_height/2]  BrickDimensionsUnits=m  ExportEntireGeometry=off  InertiaType=CalculateFromGeometry  BasedOnType=Mass  Density=1000  DensityUnits=kg/m^3  Mass=body_mass  MassUnits=kg  CenterOfMass=[0 0 0]  CenterOfMassUnits=m  MomentsOfInertia=[1 1 1]  MomentsOfInertiaUnits=kg*m^2  ProductsOfInertia=[0 0 0]  ProductsOfInertiaUnits=kg*m^2  GraphicType=FromGeometry  MarkerShape=Sphere  MarkerSize=10  GraphicVisPropType=SimpleVisualProperties  GraphicDiffuseColor=[0.8 0.8 0.8]  GraphicOpacity=1.0  GraphicSpecularColor=[0.5 0.5 0.5 1.0]  GraphicAmbientColor=[0.15 0.15 0.15 1.0]  GraphicEmissiveColor=[0.0 0.0 0.0 1.0]  GraphicShininess=75  DoExposeReferenceFrame=off  SerializedFrames=<Frames><Frame><Id>Frame1</Id><Value><Name>B</Name><Origin><Source>GeometricFeature</Source><FeatureName>-z surface</FeatureName></Origin><PrimaryAxis><DefinedDirection>+Z</DefinedDirection><Source>ReferenceFrame</Source><SourceDirection>+Z</SourceDirection><FeatureName></FeatureName></PrimaryAxis><SecondaryAxis><DefinedDirection>+X</DefinedDirection><Source>ReferenceFrame</Source><SourceDirection>+X</SourceDirection><FeatureName></FeatureName></SecondaryAxis></Value></Frame></Frames>
  Gain : Gain  Gain=-1
  Gain1 : Gain  Gain=-1
  Track L : sm_tracked_vehicle_belt_lib/Track Two Idlers  cyl_radius=cyl_radius  cyl_density=cyl_density  cyl_color_custom=cyl_color_custom  cyl_opacity=cyl_opacity  link_len=link_len  link_xlen=link_xlen  link_height=link_height  link_rado=link_rado  link_width=link_width  link_mass=link_mass  link_opc=link_opc  link_color=link_color  CoordinatesMatrix=CoordinatesMatrix  GraphicSphereRadius=GraphicSphereRadius  GraphicOpacity=GraphicOpacity  GraphicDiffuseColor=GraphicDiffuseColor
  Track R : sm_tracked_vehicle_belt_lib/Track Two Idlers  cyl_radius=cyl_radius  cyl_density=cyl_density  cyl_color_custom=cyl_color_custom  cyl_opacity=cyl_opacity  link_len=link_len  link_xlen=link_xlen  link_height=link_height  link_rado=link_rado  link_width=link_width  link_mass=link_mass  link_opc=link_opc  link_color=link_color  CoordinatesMatrix=CoordinatesMatrix  GraphicSphereRadius=GraphicSphereRadius  GraphicOpacity=GraphicOpacity  GraphicDiffuseColor=GraphicDiffuseColor
  Transform Ref : sm_lib/Frames and Transforms/Rigid Transform  RotationMethod=None  FollAlignAxisA=+X  BaseAlignAxisA=+Y  FollAlignAxisB=+Y  BaseAlignAxisB=+Z  RotationStandardAxis=+Z  RotationAngle=0  RotationAngleUnits=deg  RotationArbitraryAxis=[0 0 1]  RotationSequenceAxes=FollowerAxes  RotationSequence=XYX  RotationSequenceAngles=[0 0 0]  RotationSequenceAnglesUnits=deg  RotationMatrix=[1 0 0;0 1 0;0 0 1]  Quaternion=[1 0 0 0]  TranslationMethod=StandardAxis  TranslationCartesianOffset=[0 0 0]  TranslationCartesianOffsetUnits=m  TranslationStandardAxis=+Z  TranslationStandardOffset=-link_rado  TranslationStandardOffsetUnits=m  TranslationROffset=0  TranslationROffsetUnits=m  TranslationThetaOffset=0  TranslationThetaOffsetUnits=deg  TranslationZOffset=0  TranslationZOffsetUnits=m
  Transform Track L CG : sm_lib/Frames and Transforms/Rigid Transform  RotationMethod=None  FollAlignAxisA=+X  BaseAlignAxisA=+Y  FollAlignAxisB=+Y  BaseAlignAxisB=+Z  RotationStandardAxis=+Z  RotationAngle=0.0  RotationAngleUnits=deg  RotationArbitraryAxis=[0 0 1]  RotationSequenceAxes=FollowerAxes  RotationSequence=XYX  RotationSequenceAngles=[0 0 0]  RotationSequenceAnglesUnits=deg  RotationMatrix=[1 0 0; 0 1 0; 0 0 1]  Quaternion=[1 0 0 0]  TranslationMethod=StandardAxis  TranslationCartesianOffset=[0 0 0]  TranslationCartesianOffsetUnits=m  TranslationStandardAxis=+Y  TranslationStandardOffset=track_sep/2  TranslationStandardOffsetUnits=m  TranslationROffset=0  TranslationROffsetUnits=m  TranslationThetaOffset=0  TranslationThetaOffsetUnits=deg  TranslationZOffset=0  TranslationZOffsetUnits=m
  Transform Track R CG : sm_lib/Frames and Transforms/Rigid Transform  RotationMethod=None  FollAlignAxisA=+X  BaseAlignAxisA=+Y  FollAlignAxisB=+Y  BaseAlignAxisB=+Z  RotationStandardAxis=+Z  RotationAngle=0.0  RotationAngleUnits=deg  RotationArbitraryAxis=[0 0 1]  RotationSequenceAxes=FollowerAxes  RotationSequence=XYX  RotationSequenceAngles=[0 0 0]  RotationSequenceAnglesUnits=deg  RotationMatrix=[1 0 0; 0 1 0; 0 0 1]  Quaternion=[1 0 0 0]  TranslationMethod=StandardAxis  TranslationCartesianOffset=[0 0 0]  TranslationCartesianOffsetUnits=m  TranslationStandardAxis=+Y  TranslationStandardOffset=track_sep/2  TranslationStandardOffsetUnits=m  TranslationROffset=0  TranslationROffsetUnits=m  TranslationThetaOffset=0  TranslationThetaOffsetUnits=deg  TranslationZOffset=0  TranslationZOffsetUnits=m
  w to spd L : Gain  Gain=link_rado
  w to spd R : Gain  Gain=link_rado
  PCR : PMIOPort  Side=Right
  PCL : PMIOPort  Port=2  Side=Right
  Ref : PMIOPort  Port=3  Side=Right
  vxR : Outport
  vxL : Outport  Port=2
  wires:
  Spd R/1 -> Track R/1, w to spd R/1
  Spd L/1 -> Track L/1, w to spd L/1
  w to spd R/1 -> Gain1/1  "vx"
  w to spd L/1 -> Gain/1  "vx"
  Gain/1 -> vxL/1
  Gain1/1 -> vxR/1
  connections:
  Track R/RConn1 -- Transform Track R CG/LConn1
  Track L/RConn1 -- Transform Track L CG/RConn1
  Transform Track L CG/LConn1 -- Transform Ref/LConn1 -- Body/LConn1 -- Transform Track R CG/RConn1
  Track R/RConn2 -- PCR/RConn1
  Track L/RConn2 -- PCL/RConn1
  Ref/RConn1 -- Transform Ref/RConn1
